simulink model "TempControl_Simulation"  (R2026b)
settings: Solver=VariableStepAuto  StopTime=600
values from neighbouring files (symbols this model uses):
  K = p(1)    [prep_lab_1.m]
  T0 = mean(T(t < t_step & t > t_step - 20))    [prep_lab_1.m]
  t_step = t(idx)    [prep_lab_1.m]
  tau = p(2)    [prep_lab_1.m]
  Tt = p(3)    [prep_lab_1.m]
settings Model: Creator=ursmu  LastModifiedBy=ursmu

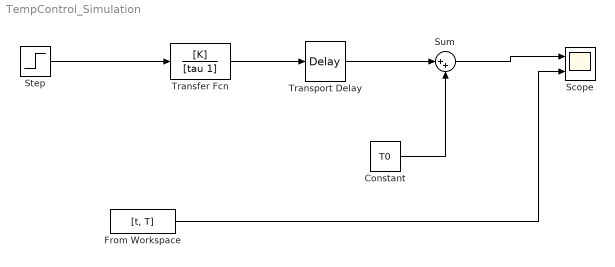
== system TempControl_Simulation ==
  Constant : Constant  Value=T0
  From Workspace : FromWorkspace  VariableName=[t, T]
  Scope : Scope  NumInputPorts=2
      settings: ActiveDisplayYMinimum=23.615698030254563  ActiveDisplayYMaximum=32.92147399408892
  Step : Step  Time=t_step  FinalValue=dD  SampleTime=0
  Sum : Sum  Inputs=|++
  Transfer Fcn : TransferFcn  Numerator=[K]  Denominator=[tau 1]
  Transport Delay : TransportDelay  DelayTime=Tt
  wires:
  Step/1 -> Transfer Fcn/1
  Transfer Fcn/1 -> Transport Delay/1
  Constant/1 -> Sum/2
  Transport Delay/1 -> Sum/1
  Sum/1 -> Scope/1
  From Workspace/1 -> Scope/2
